simulink model "Twin_Builder"  (R2026a)
settings: Solver=VariableStepAuto  StopTime=simTime  FixedStep=Ts/60  RelTol=1e-2
values from neighbouring files (symbols this model uses):
  ac = log(9)/tr    [Run_Twin.m]
  as = 0.08 * ac    [Run_Twin.m]
  ath = 0.25 * as    [Run_Twin.m]
  B = 0.00001    (= 1e-05)    [Run_Twin.m]
  BEMFD_FEA_PerHz = InterpFEA_Data_ForSimulink(FEA_Data.BackEMFD_perHz, IS_FEA, IEA_FEA, IS_Interp, IEA_Interp)    [Run_Twin.m]
  BEMFQ_FEA_PerHz = InterpFEA_Data_ForSimulink(FEA_Data.BackEMFQ_perHz, IS_FEA, IEA_FEA, IS_Interp, IEA_Interp)    [Run_Twin.m]
  CondLoss_Inv = zeros([length(IS_Interp), size(FEA_Data.ConductionLoss, [2 3] ) ])    [Run_Twin.m]
  CopperLoss_FEA = InterpFEA_Data_ForSimulink(FEA_Data.CopperLosses, IS_FEA, IEA_FEA, IS_Interp, IEA_Interp)    [Run_Twin.m]
  DriveMethod = 1    [Run_Twin.m]
  EnvTorque_FW = interp1(Speed_full, Env_full, Speed_Vec, 'pchip', 'extrap')    [Run_Twin.m]
  f_sw = 10e3    (= 10000)    [Run_Twin.m]
  FEA_Data = LoadData.(FieldData{1})    [Run_Twin.m]
  FILTER_COEFF = 0.23    [Run_Twin.m]
  FluxD_FEA = InterpFEA_Data_ForSimulink(FEA_Data.FluxD, IS_FEA, IEA_FEA, IS_Interp, IEA_Interp)    [Run_Twin.m]
  FluxQ_FEA = InterpFEA_Data_ForSimulink(FEA_Data.FluxQ, IS_FEA, IEA_FEA, IS_Interp, IEA_Interp)    [Run_Twin.m]
  FrictLoss_FEA = squeeze( FEA_Data.FrictLosses(1,1,:) )    [Run_Twin.m]
  GateLoss_Inv = zeros([length(IS_Interp), size(FEA_Data.ConductionLoss, [2 3] ) ])    [Run_Twin.m]
  IDcore_FEA = InterpFEA_Data_ForSimulink(FEA_Data.IDc, IS_FEA, IEA_FEA, IS_Interp, IEA_Interp)    [Run_Twin.m]
  IEA_FEA = IEA_Interp    [Run_Twin.m]
  IQcore_FEA = InterpFEA_Data_ForSimulink(FEA_Data.IQc, IS_FEA, IEA_FEA, IS_Interp, IEA_Interp)    [Run_Twin.m]
  IronLoss_FEA = InterpFEA_Data_ForSimulink(FEA_Data.IronLosses,   IS_FEA, IEA_FEA, IS_Interp, IEA_Interp)    [Run_Twin.m]
  Is_Amp = 40    [Run_Twin.m]
  IS_FEA = IS_Interp    [Run_Twin.m]
  J = FEA_Data.Jinertia    [Run_Twin.m]
  J_Control = FEA_Data.Jinertia    [Run_Twin.m]
  LD_FEA = InterpFEA_Data_ForSimulink(FEA_Data.LD, IS_FEA, IEA_FEA, IS_Interp, IEA_Interp)    [Run_Twin.m]
  LD_Single = mean(LD_FEA, 'all')    [Run_Twin.m]
  LQ_FEA = InterpFEA_Data_ForSimulink(FEA_Data.LQ, IS_FEA, IEA_FEA, IS_Interp, IEA_Interp)    [Run_Twin.m]
  LQ_Single = mean(LQ_FEA, 'all')    [Run_Twin.m]
  MagnetLoss_FEA = InterpFEA_Data_ForSimulink(FEA_Data.MagnetLosses, IS_FEA, IEA_FEA, IS_Interp, IEA_Interp)    [Run_Twin.m]
  MaxSpeed = max(Speed_Vec)    [Run_Twin.m]
  MaxTe = max(Torque_FEA, [], 'all')    [Run_Twin.m]
  ModStrategy = 1    [Run_Twin.m]
  PMFlux_FEA = interp1(IS_FEA, squeeze( FEA_Data.FluxD(:,IEA_FEA == 90, :) ), IS_Interp, 'pchip' )    [Run_Twin.m]
  PMFlux_Single = mean( PMFlux_FEA, 'all' )    [Run_Twin.m]
  PMT_ID = round( F_ID(PMT_grid, Speed_grid), 2)    [Run_Twin.m]
  PMT_IQ = round( F_IQ(PMT_grid, Speed_grid), 2)    [Run_Twin.m]
  PMT_Vec = linspace(0,   100,   InterpSamples)    [Run_Twin.m]
  PolePair = FEA_Data.Poles / 2    [Run_Twin.m]
  PPR = 1024    [Run_Twin.m]
  ProxiLoss_FEA = InterpFEA_Data_ForSimulink(FEA_Data.ProxiLosses,  IS_FEA, IEA_FEA, IS_Interp, IEA_Interp)    [Run_Twin.m]
  Rcore_FEA = InterpFEA_Data_ForSimulink(FEA_Data.Rcore, IS_FEA, IEA_FEA, IS_Interp, IEA_Interp)    [Run_Twin.m]
  RDC = squeeze( Rseries_FEA(1,1,1) )    [Run_Twin.m]
  RefSpeed = [50, 400, 250, 500, 400]    [Run_Twin.m]
  RefTheta = [50, 0, 140, 300, -50]    [Run_Twin.m]
  Rseries_FEA = InterpFEA_Data_ForSimulink(FEA_Data.Rs,    IS_FEA, IEA_FEA, IS_Interp, IEA_Interp)    [Run_Twin.m]
  ShafthLoad = [10, 25, 3, 8, 10]    [Run_Twin.m]
  simTime = mechThetaTarget / wMechTarget    [Run_Twin.m]
  Speed_FEA = FEA_Data.Speed_vec    [Run_Twin.m]
  Speed_Vec = linspace(min(Speed_full), max(Speed_full), InterpSamples)    [Run_Twin.m]
  speedTarget = 200    [Run_Twin.m]
  SR_FEA = FEA_Data.SynchAngle    [Run_Twin.m]
  SwitchLoss_Inv = zeros([length(IS_Interp), size(FEA_Data.ConductionLoss, [2 3] ) ])    [Run_Twin.m]
  Tdt = 0.3 * 1e-6    (= 3e-07)    [Run_Twin.m]
  Throttle = 45    [Run_Twin.m]
  Times = [0, 0.2, 0.4, 0.6, 0.8] * simTime    [Run_Twin.m]
  Torque_FEA = InterpFEA_Data_ForSimulink(FEA_Data.TorqueFEA, IS_FEA, IEA_FEA, IS_Interp, IEA_Interp)    [Run_Twin.m]
  Ts = 1/f_sw    (= 0.0001)    [Run_Twin.m]
  Ts_Sp = 2 * Ts    (= 0.0002)    [Run_Twin.m]
  Vdc = 56    [Run_Twin.m]
  Vs_pu = 0.98    [Run_Twin.m]
  WindageLoss_FEA = squeeze( FEA_Data.WindLosses(1,1,:) )    [Run_Twin.m]
undefined symbols (not defined in the file or in its folder): DiscIntNeverNeededParam, feNom, mf, OverMod, PMT_Speed, SimData, Tables
libraries: simulink x14, ee_lib x11, simulink_extras x7, eeTransforms x6, fl_lib x6, eeGeneralControl x4, spsMeanLib x2, dspxfrm3 x1
(part 2 of 3)

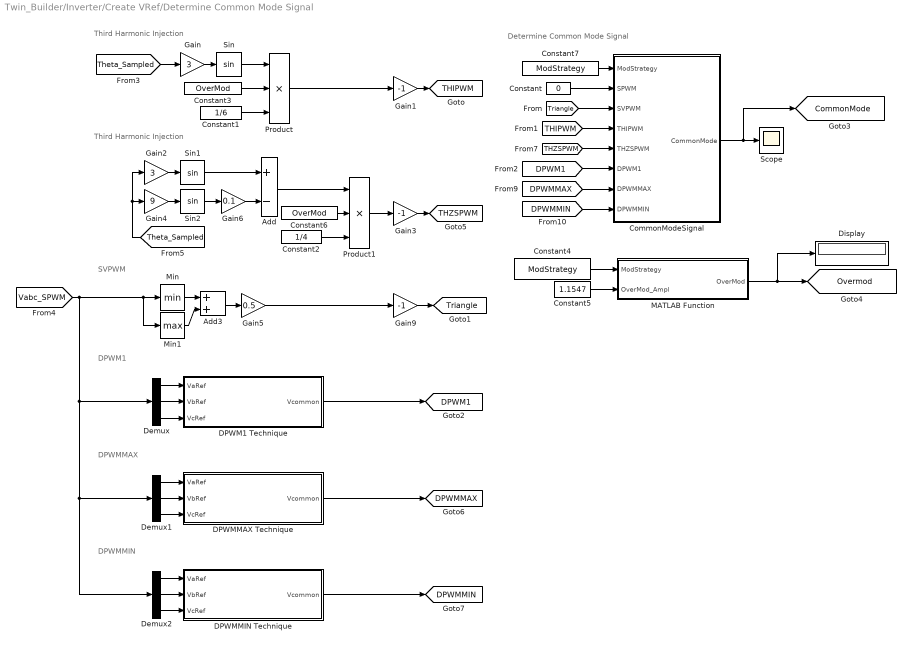
== system Twin_Builder/Inverter/Create VRef/Determine Common Mode Signal ==
  note: SVPWM
  note: Third Harmonic Injection
  note: Determine Common Mode Signal
  note: DPWM1
  note: Third Harmonic Injection
  note: DPWMMAX
  note: DPWMMIN
  Add : Sum  Inputs=+-
  Add3 : Sum
  CommonModeSignal : MATLAB Function  TreatAsAtomicUnit=on
  Constant : Constant  Value=0
  Constant1 : Constant  Value=1/6  SampleTime=0
  Constant2 : Constant  Value=1/4  SampleTime=0
  Constant3 : Constant  Value=OverMod  SampleTime=0
  Constant4 : Constant  Value=ModStrategy  SampleTime=0
  Constant5 : Constant  Value=1.1547  SampleTime=0
  Constant6 : Constant  Value=OverMod  SampleTime=0
  Constant7 : Constant  Value=ModStrategy  SampleTime=0
  DPWM1 Technique : MATLAB Function  TreatAsAtomicUnit=on
  DPWMMAX Technique : MATLAB Function  TreatAsAtomicUnit=on
  DPWMMIN Technique : MATLAB Function  TreatAsAtomicUnit=on
  Demux : Demux  Outputs=3
  Demux1 : Demux  Outputs=3
  Demux2 : Demux  Outputs=3
  Display : Display
  Gain : Gain  Gain=3
  Gain1 : Gain  Gain=-1
  Gain2 : Gain  Gain=3
  Gain3 : Gain  Gain=-1
  Gain4 : Gain  Gain=9
  Gain5 : Gain  Gain=0.5
  Gain6 : Gain  Gain=0.1
  Gain9 : Gain  Gain=-1
  MATLAB Function : MATLAB Function  TreatAsAtomicUnit=on
  Min : MinMax
  Min1 : MinMax  Function=max
  Product : Product  Inputs=3
  Product1 : Product  Inputs=3
  Scope : Scope
      settings: ActiveDisplayYMinimum=-0.35295  ActiveDisplayYMaximum=0.35321
  Sin : Trigonometry
  Sin1 : Trigonometry
  Sin2 : Trigonometry
  tag scope: CommonMode=global, DPWM1=global, DPWMMAX=global, DPWMMIN=global, Overmod=global, THIPWM=global, THZSPWM=global, Triangle=global
  wires:
  Constant/1 -> CommonModeSignal/2(SPWM)
  Min/1 -> Add3/1
  Gain9/1 -> [Triangle]
  Gain5/1 -> Gain9/1
  Add3/1 -> Gain5/1
  Min1/1 -> Add3/2
  Constant7/1 -> CommonModeSignal/1(ModStrategy)
  [Triangle] -> CommonModeSignal/3(SVPWM)
  [THIPWM] -> CommonModeSignal/4(THIPWM)
  DPWM1 Technique/1(Vcommon) -> [DPWM1]
  Demux/1 -> DPWM1 Technique/1(VaRef)
  Demux/2 -> DPWM1 Technique/2(VbRef)
  Demux/3 -> DPWM1 Technique/3(VcRef)
  CommonModeSignal/1(CommonMode) -> [CommonMode], Scope/1
  [Theta_Sampled] -> Gain/1
  Gain/1 -> Sin/1
  Sin/1 -> Product/1
  Constant3/1 -> Product/2
  Constant1/1 -> Product/3
  Product/1 -> Gain1/1
  Constant4/1 -> MATLAB Function/1(ModStrategy)
  Constant5/1 -> MATLAB Function/2(OverMod_Ampl)
  MATLAB Function/1(OverMod) -> Display/1, [Overmod]
  Gain1/1 -> [THIPWM]
  Gain2/1 -> Sin1/1
  [Theta_Sampled] -> Gain2/1, Gain4/1
  Constant6/1 -> Product1/2
  Gain4/1 -> Sin2/1
  Product1/1 -> Gain3/1
  Gain3/1 -> [THZSPWM]
  Sin2/1 -> Gain6/1
  Sin1/1 -> Add/1
  Gain6/1 -> Add/2
  Add/1 -> Product1/1
  [DPWM1] -> CommonModeSignal/6(DPWM1)
  [THZSPWM] -> CommonModeSignal/5(THZSPWM)
  Constant2/1 -> Product1/3
  DPWMMAX Technique/1(Vcommon) -> [DPWMMAX]
  Demux1/1 -> DPWMMAX Technique/1(VaRef)
  Demux1/2 -> DPWMMAX Technique/2(VbRef)
  Demux1/3 -> DPWMMAX Technique/3(VcRef)
  [DPWMMAX] -> CommonModeSignal/7(DPWMMAX)
  [DPWMMIN] -> CommonModeSignal/8(DPWMMIN)
  Demux2/1 -> DPWMMIN Technique/1(VaRef)
  Demux2/3 -> DPWMMIN Technique/3(VcRef)
  Demux2/2 -> DPWMMIN Technique/2(VbRef)
  DPWMMIN Technique/1(Vcommon) -> [DPWMMIN]
  [Vabc_SPWM] -> Demux/1, Demux1/1, Demux2/1, Min1/1, Min/1

== system Twin_Builder/Inverter/Create VRef/Finalize References ==
  note: Wrap References to [0,1] and saturate them
  Vabc_Ref : Inport
  Add : Sum
  Constant1 : Constant  Value=0  SampleTime=0
  Constant2 : Constant  Value=0.5  SampleTime=0
  Constant3 : Constant  SampleTime=0
  Demux : Demux  Outputs=3
  Divide1 : Product  Inputs=*/
  Gain3 : Gain  Gain=0.5
  Max : MinMax  Function=max  Inputs=4
  Max1 : MinMax  Function=max  Inputs=2
  Vabc_Ref_Final : Outport
  wires:
  Constant2/1 -> Add/2
  Gain3/1 -> Add/1
  Vabc_Ref/1 -> Gain3/1
  Demux/3 -> Max/3
  Constant3/1 -> Max/4
  Demux/1 -> Max/1
  Demux/2 -> Max/2
  Max/1 -> Divide1/2
  Add/1 -> Divide1/1, Demux/1
  Divide1/1 -> Max1/1
  Max1/1 -> Vabc_Ref_Final/1
  Constant1/1 -> Max1/2

== system Twin_Builder/PMSM /LUTS/QEP  ==
  theta : Inport
  Abs1 : Abs  SaturateOnIntegerOverflow=off
  Constant1 : Constant  Value=PolePair
  Constant3 : Constant  Value=Ts_Sp
  Constant5 : Constant  Value=PolePair
  Constant6 : Constant  Value=FILTER_COEFF
  Constant8 : Constant  Value=PPR
  Divide2 : Product  Inputs=*/
  Product : Product
  "Quantize Electrical Theta " : MATLAB Function  TreatAsAtomicUnit=on
  Sample θ : MATLAB Function  TreatAsAtomicUnit=on
  Scope : Scope
      settings: ActiveDisplayYMinimum=-0.78520641579896233  ActiveDisplayYMaximum=7.0668577421906633
  Terminator1 : Terminator
  Terminator2 : Terminator
  omega2rpm2 : Gain  Gain=60/(2*pi)
  theta_sampled : Outport
  Omegae : Outport  Port=2
  Speed : Outport  Port=3
  wires:
  omega2rpm2/1 -> Abs1/1
  Constant6/1 -> Sample θ/3(FILTER_COEFF)
  Abs1/1 -> Speed/1
  Sample θ/2(delta_theta) -> Terminator2/1
  Constant3/1 -> Sample θ/2(Ts)
  Constant1/1 -> Divide2/2
  Sample θ/1(omega) -> Divide2/1
  Divide2/1 -> Product/2, omega2rpm2/1
  Constant8/1 -> "Quantize Electrical Theta "/2(PPR)
  theta/1 -> "Quantize Electrical Theta "/1(theta_w)
  "Quantize Electrical Theta "/2(Count) -> Terminator1/1
  "Quantize Electrical Theta "/1(Theta_mcu) -> Scope/1, theta_sampled/1, Sample θ/1(theta)
  Constant5/1 -> Product/1
  Product/1 -> Omegae/1

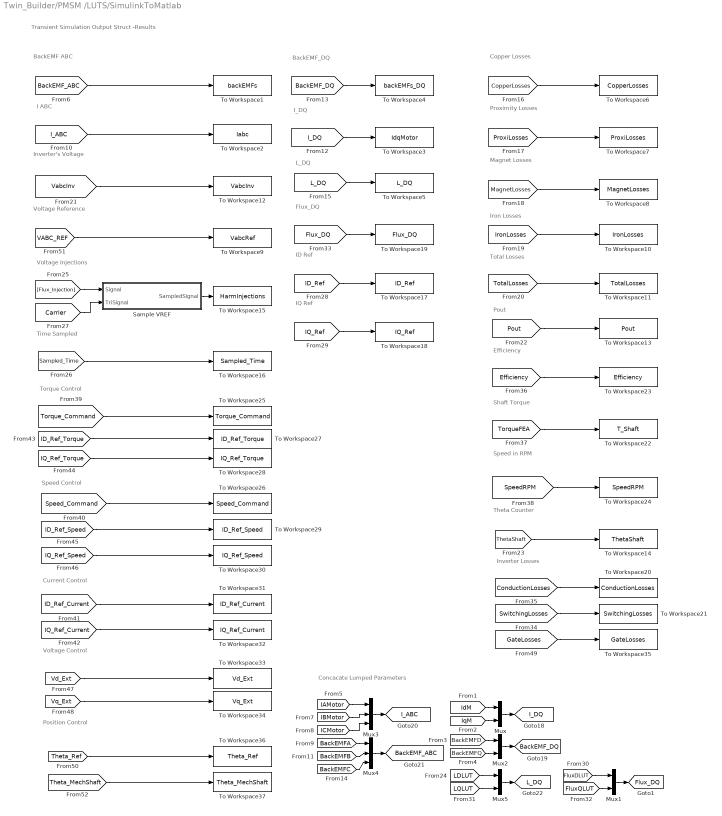
== system Twin_Builder/PMSM /LUTS/SimulinkToMatlab ==
  note: Voltage Reference
  note: Transient Simulation Output Struct -Results
  note: BackEMF ABC
  note: I_DQ
  note: BackEMF_DQ
  note: L_DQ
  note: Copper Losses
  note: Proximity Losses
  note: Magnet Losses
  note: Iron Losses
  note: Total Losses
  note: Inverter's Voltage
  note: Pout
  note: Theta Counter
  note: Voltage Injections
  note: Time Sampled
  note: ID Ref
  note: IQ Ref
  note: Efficiency
  note: Concacate Lumped Parameters
  note: I ABC
  note: Flux_DQ
  note: Inverter Losses
  note: Shaft Torque
  note: Speed in RPM
  note: Torque Control
  note: Speed Control
  note: Current Control
  note: Voltage Control
  note: Position Control
  Mux{,1..2,5} (4 alike) : Mux  Inputs=2
  Mux3 : Mux  Inputs=3
  Mux4 : Mux  Inputs=3
  Sample VREF : MATLAB Function  TreatAsAtomicUnit=on
  To Workspace1 : ToWorkspace  VariableName=backEMFs  SampleTime=-1
  To Workspace10 : ToWorkspace  VariableName=IronLosses  SampleTime=-1
  To Workspace11 : ToWorkspace  VariableName=TotalLosses  SampleTime=-1
  To Workspace12 : ToWorkspace  VariableName=VabcInv  SampleTime=-1
  To Workspace13 : ToWorkspace  VariableName=Pout  SampleTime=-1
  To Workspace14 : ToWorkspace  VariableName=ThetaShaft  SampleTime=-1
  To Workspace15 : ToWorkspace  VariableName=HarmInjections  SampleTime=-1
  To Workspace16 : ToWorkspace  VariableName=Sampled_Time  SampleTime=-1
  To Workspace17 : ToWorkspace  VariableName=ID_Ref  SampleTime=-1
  To Workspace18 : ToWorkspace  VariableName=IQ_Ref  SampleTime=-1
  To Workspace19 : ToWorkspace  VariableName=Flux_DQ  SampleTime=-1
  To Workspace2 : ToWorkspace  VariableName=Iabc  SampleTime=-1
  To Workspace20 : ToWorkspace  VariableName=ConductionLosses  SampleTime=-1
  To Workspace21 : ToWorkspace  VariableName=SwitchingLosses  SampleTime=-1
  To Workspace22 : ToWorkspace  VariableName=T_Shaft  SampleTime=-1
  To Workspace23 : ToWorkspace  VariableName=Efficiency  SampleTime=-1
  To Workspace24 : ToWorkspace  VariableName=SpeedRPM  SampleTime=-1
  To Workspace25 : ToWorkspace  VariableName=Torque_Command  SampleTime=-1
  To Workspace26 : ToWorkspace  VariableName=Speed_Command  SampleTime=-1
  To Workspace27 : ToWorkspace  VariableName=ID_Ref_Torque  SampleTime=-1
  To Workspace28 : ToWorkspace  VariableName=IQ_Ref_Torque  SampleTime=-1
  To Workspace29 : ToWorkspace  VariableName=ID_Ref_Speed  SampleTime=-1
  To Workspace3 : ToWorkspace  VariableName=IdqMotor  SampleTime=-1
  To Workspace30 : ToWorkspace  VariableName=IQ_Ref_Speed  SampleTime=-1
  To Workspace31 : ToWorkspace  VariableName=ID_Ref_Current  SampleTime=-1
  To Workspace32 : ToWorkspace  VariableName=IQ_Ref_Current  SampleTime=-1
  To Workspace33 : ToWorkspace  VariableName=Vd_Ext  SampleTime=-1
  To Workspace34 : ToWorkspace  VariableName=Vq_Ext  SampleTime=-1
  To Workspace35 : ToWorkspace  VariableName=GateLosses  SampleTime=-1
  To Workspace36 : ToWorkspace  VariableName=Theta_Ref  SampleTime=-1
  To Workspace37 : ToWorkspace  VariableName=Theta_MechShaft  SampleTime=-1
  To Workspace4 : ToWorkspace  VariableName=backEMFs_DQ  SampleTime=-1
  To Workspace5 : ToWorkspace  VariableName=L_DQ  SampleTime=-1
  To Workspace6 : ToWorkspace  VariableName=CopperLosses  SampleTime=-1
  To Workspace7 : ToWorkspace  VariableName=ProxiLosses  SampleTime=-1
  To Workspace8 : ToWorkspace  VariableName=MagnetLosses  SampleTime=-1
  To Workspace9 : ToWorkspace  VariableName=VabcRef  SampleTime=-1
  tag scope: BackEMF_ABC=global, BackEMF_DQ=global, Flux_DQ=global, I_ABC=global, I_DQ=global, L_DQ=global
  wires:
  [ThetaShaft] -> To Workspace14/1
  [BackEMF_DQ] -> To Workspace4/1
  [VabcInv] -> To Workspace12/1
  [I_DQ] -> To Workspace3/1
  [Efficiency] -> To Workspace23/1
  [CopperLosses] -> To Workspace6/1
  [BackEMF_ABC] -> To Workspace1/1
  [VABC_REF] -> To Workspace9/1
  [MagnetLosses] -> To Workspace8/1
  [ProxiLosses] -> To Workspace7/1
  [Flux_Injection] -> Sample VREF/1(Signal)
  Sample VREF/1(SampledSignal) -> To Workspace15/1
  [Pout] -> To Workspace13/1
  [TotalLosses] -> To Workspace11/1
  [IQ_Ref] -> To Workspace18/1
  [Carrier] -> Sample VREF/2(TriSignal)
  [IronLosses] -> To Workspace10/1
  [ID_Ref] -> To Workspace17/1
  [L_DQ] -> To Workspace5/1
  [Sampled_Time] -> To Workspace16/1
  [BackEMFC] -> Mux4/3
  [BackEMFA] -> Mux4/1
  Mux4/1 -> [BackEMF_ABC]
  [BackEMFB] -> Mux4/2
  [LQLUT] -> Mux5/2
  Mux3/1 -> [I_ABC]
  Mux/1 -> [I_DQ]
  [LDLUT] -> Mux5/1
  [IdM] -> Mux/1
  [IBMotor] -> Mux3/2
  [IAMotor] -> Mux3/1
  [ICMotor] -> Mux3/3
  Mux5/1 -> [L_DQ]
  [IqM] -> Mux/2
  Mux2/1 -> [BackEMF_DQ]
  [BackEMFQ] -> Mux2/2
  [BackEMFD] -> Mux2/1
  [I_ABC] -> To Workspace2/1
  [FluxDLUT] -> Mux1/1
  Mux1/1 -> [Flux_DQ]
  [FluxQLUT] -> Mux1/2
  [Flux_DQ] -> To Workspace19/1
  [ConductionLosses] -> To Workspace20/1
  [SwitchingLosses] -> To Workspace21/1
  [TorqueFEA] -> To Workspace22/1
  [SpeedRPM] -> To Workspace24/1
  [Torque_Command] -> To Workspace25/1
  [Speed_Command] -> To Workspace26/1
  [ID_Ref_Torque] -> To Workspace27/1
  [IQ_Ref_Torque] -> To Workspace28/1
  [ID_Ref_Speed] -> To Workspace29/1
  [IQ_Ref_Speed] -> To Workspace30/1
  [ID_Ref_Current] -> To Workspace31/1
  [IQ_Ref_Current] -> To Workspace32/1
  [Vd_Ext] -> To Workspace33/1
  [Vq_Ext] -> To Workspace34/1
  [GateLosses] -> To Workspace35/1
  [Theta_Ref] -> To Workspace36/1
  [Theta_MechShaft] -> To Workspace37/1

== system Twin_Builder/PMSM /LUTS/TorqueInduced from Fluxes ==
  note: Torque with Fluxes
  Gain1 : Gain  Gain=3*PolePair/2
  Product3 : Product
  Product4 : Product
  Sum2 : Sum  Inputs=|+-
  tag scope: Te=global
  wires:
  [FluxDLUT] -> Product3/1
  [IqM] -> Product3/2
  [FluxQLUT] -> Product4/1
  [IdM] -> Product4/2
  Product3/1 -> Sum2/1
  Product4/1 -> Sum2/2
  Sum2/1 -> Gain1/1
  Gain1/1 -> [Te]

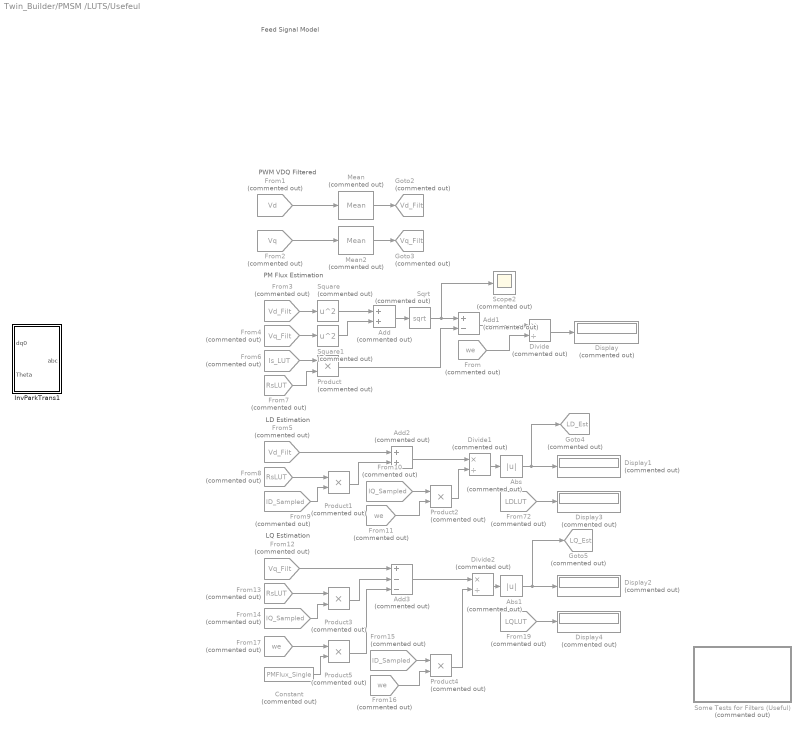
== system Twin_Builder/PMSM /LUTS/Usefeul ==
  note: PM Flux Estimation
  note: PWM VDQ Filtered
  note: LD Estimation
  note: LQ Estimation
  note: Feed Signal Model
  Abs : Abs  Commented=on  SaturateOnIntegerOverflow=off
  Abs1 : Abs  Commented=on  SaturateOnIntegerOverflow=off
  Add : Sum  Commented=on
  Add1 : Sum  Commented=on  Inputs=+-
  Add2 : Sum  Commented=on
  Add3 : Sum  Commented=on  Inputs=+--
  Constant : Constant  Commented=on  Value=PMFlux_Single  SampleTime=0
  Display{,1..4} (5 alike) : Display  Commented=on
  Divide : Product  Commented=on  Inputs=*/
  Divide1 : Product  Commented=on  Inputs=*/
  Divide2 : Product  Commented=on  Inputs=*/
  From{,11,16..17} (4 alike) : From  Commented=on  GotoTag=we  TagVisibility=global
  From1 : From  Commented=on  GotoTag=Vd  TagVisibility=global
  From10 : From  Commented=on  GotoTag=IQ_Sampled  TagVisibility=global
  From12 : From  Commented=on  GotoTag=Vq_Filt  TagVisibility=global
  From13 : From  Commented=on  GotoTag=RsLUT  TagVisibility=global
  From14 : From  Commented=on  GotoTag=IQ_Sampled  TagVisibility=global
  From15 : From  Commented=on  GotoTag=ID_Sampled  TagVisibility=global
  From19 : From  Commented=on  GotoTag=LQLUT  TagVisibility=global
  From2 : From  Commented=on  GotoTag=Vq  TagVisibility=global
  From3 : From  Commented=on  GotoTag=Vd_Filt  TagVisibility=global
  From4 : From  Commented=on  GotoTag=Vq_Filt  TagVisibility=global
  From5 : From  Commented=on  GotoTag=Vd_Filt  TagVisibility=global
  From6 : From  Commented=on  GotoTag=Is_LUT  TagVisibility=global
  From7 : From  Commented=on  GotoTag=RsLUT  TagVisibility=global
  From72 : From  Commented=on  GotoTag=LDLUT  TagVisibility=global
  From8 : From  Commented=on  GotoTag=RsLUT  TagVisibility=global
  From9 : From  Commented=on  GotoTag=ID_Sampled  TagVisibility=global
  Goto2 : Goto  Commented=on  GotoTag=Vd_Filt  TagVisibility=global
  Goto3 : Goto  Commented=on  GotoTag=Vq_Filt  TagVisibility=global
  Goto4 : Goto  Commented=on  GotoTag=LD_Est  TagVisibility=global
  Goto5 : Goto  Commented=on  GotoTag=LQ_Est  TagVisibility=global
  InvParkTrans1 : Subsystem
  Mean : spsMeanLib/Mean  Commented=on  Freq=60  Vinit=0  Ts=0
  Mean2 : spsMeanLib/Mean  Commented=on  Freq=60  Vinit=0  Ts=0
  Product{,1..5} (6 alike) : Product  Commented=on
  Scope2 : Scope  Commented=on
      settings: ActiveDisplayYMinimum=-0.82581  ActiveDisplayYMaximum=7.43229
  Some Tests for Filters (Useful) : Subsystem  Commented=on
  Sqrt : Sqrt  Commented=on
  Square : Math  Commented=on  Operator=square
  Square1 : Math  Commented=on  Operator=square
  wires:
  Add/1 -> Sqrt/1
  Square1/1 -> Add/2
  Square/1 -> Add/1
  From6/1 -> Product/1
  From7/1 -> Product/2
  Product/1 -> Add1/2
  Add1/1 -> Divide/1
  From/1 -> Divide/2
  Divide/1 -> Display/1
  Sqrt/1 -> Scope2/1, Add1/1
  From3/1 -> Square/1
  From4/1 -> Square1/1
  From2/1 -> Mean2/1
  From1/1 -> Mean/1
  Mean/1 -> Goto2/1
  Mean2/1 -> Goto3/1
  From5/1 -> Add2/1
  From9/1 -> Product1/2
  From8/1 -> Product1/1
  Product1/1 -> Add2/2
  From10/1 -> Product2/1
  From11/1 -> Product2/2
  Add2/1 -> Divide1/1
  Product2/1 -> Divide1/2
  Divide1/1 -> Abs/1
  From14/1 -> Product3/2
  From13/1 -> Product3/1
  From12/1 -> Add3/1
  Product3/1 -> Add3/2
  From16/1 -> Product4/2
  From15/1 -> Product4/1
  From17/1 -> Product5/1
  Constant/1 -> Product5/2
  Product5/1 -> Add3/3
  Add3/1 -> Divide2/1
  Product4/1 -> Divide2/2
  Divide2/1 -> Abs1/1
  From72/1 -> Display3/1
  From19/1 -> Display4/1
  Abs/1 -> Display1/1, Goto4/1
  Abs1/1 -> Display2/1, Goto5/1

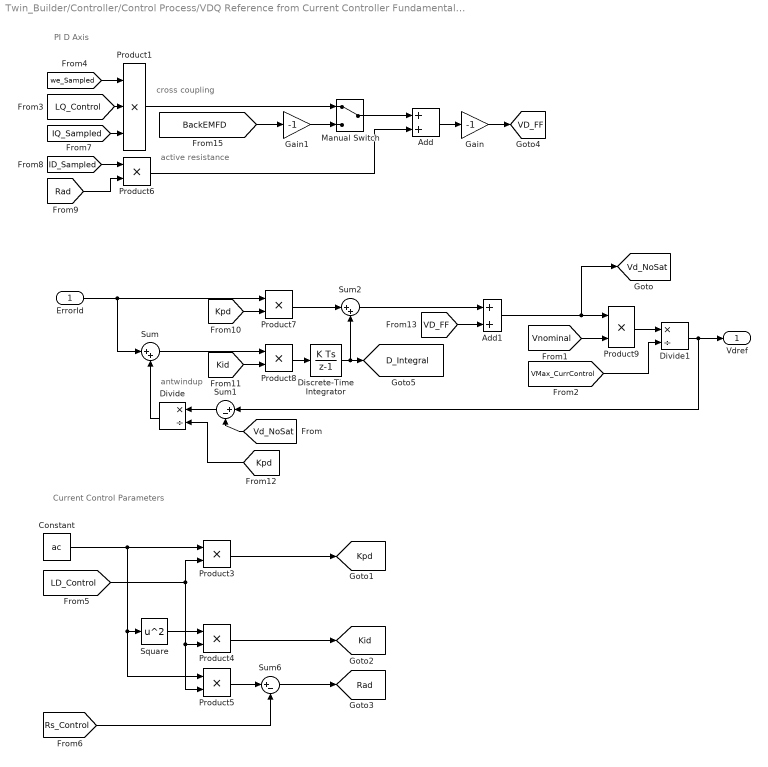
== system Twin_Builder/Controller/Control Process/VDQ Reference from Current Controller Fundamental/CurrentControlD ==
  note: active resistance
  note: cross coupling
  note: Current Control Parameters
  note: PI D Axis
  note: antwindup
  ErrorId : Inport
  Add : Sum
  Add1 : Sum
  Constant : Constant  Value=ac  SampleTime=0
  Discrete-Time Integrator : DiscreteIntegrator  SampleTime=Ts  ICPrevOutput=DiscIntNeverNeededParam  ICPrevScaledInput=DiscIntNeverNeededParam
  Divide : Product  Inputs=*/
  Divide1 : Product  Inputs=*/
  Gain : Gain  Gain=-1
  Gain1 : Gain  Gain=-1
  Manual Switch : ManualSwitch
  Product1 : Product  Inputs=3
  Product{3..9} (7 alike) : Product
  Square : Math  Operator=square
  Sum : Sum  Inputs=|++
  Sum1 : Sum  Inputs=|+-
  Sum2 : Sum  Inputs=|++
  Sum6 : Sum  Inputs=|+-
  Vdref : Outport
  tag scope: D_Integral=global, Kid=global, Kpd=global, Rad=global, VD_FF=global, Vd_NoSat=global
  wires:
  Sum/1 -> Product8/1
  Product7/1 -> Sum2/1
  ErrorId/1 -> Sum/1, Product7/1
  Product8/1 -> Discrete-Time Integrator/1
  Product6/1 -> Add/2
  Sum2/1 -> Add1/1
  Discrete-Time Integrator/1 -> [D_Integral], Sum2/2
  Product3/1 -> [Kpd]
  Square/1 -> Product4/1
  Constant/1 -> Product3/1, Product5/1, Square/1
  Product5/1 -> Sum6/1
  Sum6/1 -> [Rad]
  [Rad] -> Product6/2
  [Kpd] -> Product7/2
  [Kid] -> Product8/2
  Sum1/1 -> Divide/1
  Divide/1 -> Sum/2
  [Kpd] -> Divide/2
  Product4/1 -> [Kid]
  [Rs_Control] -> Sum6/2
  [LD_Control] -> Product3/2, Product5/2, Product4/2
  [Vnominal] -> Product9/2
  Product9/1 -> Divide1/1
  [VMax_CurrControl] -> Divide1/2
  Divide1/1 -> Vdref/1, Sum1/1
  [ID_Sampled] -> Product6/1
  [we_Sampled] -> Product1/1
  [LQ_Control] -> Product1/2
  [IQ_Sampled] -> Product1/3
  [Vd_NoSat] -> Sum1/2
  Add/1 -> Gain/1
  Gain/1 -> [VD_FF]
  Add1/1 -> [Vd_NoSat], Product9/1
  [VD_FF] -> Add1/2
  Manual Switch/1 -> Add/1
  Product1/1 -> Manual Switch/1
  [BackEMFD] -> Gain1/1
  Gain1/1 -> Manual Switch/2

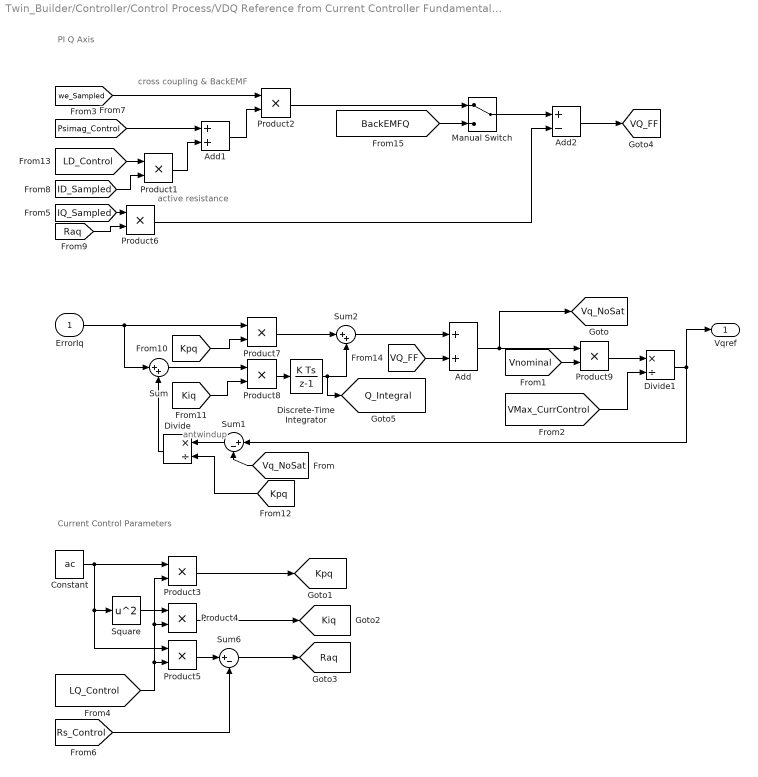
== system Twin_Builder/Controller/Control Process/VDQ Reference from Current Controller Fundamental/CurrentControlQ ==
  note: active resistance
  note: cross coupling & BackEMF
  note: Current Control Parameters
  note: PI Q Axis
  note: antwindup
  ErrorIq : Inport
  Add : Sum
  Add1 : Sum
  Add2 : Sum  Inputs=+-
  Constant : Constant  Value=ac
  Discrete-Time Integrator : DiscreteIntegrator  SampleTime=Ts  ICPrevOutput=DiscIntNeverNeededParam  ICPrevScaledInput=DiscIntNeverNeededParam
  Divide : Product  Inputs=*/
  Divide1 : Product  Inputs=*/
  Manual Switch : ManualSwitch
  Product{1..9} (9 alike) : Product
  Square : Math  Operator=square
  Sum : Sum  Inputs=|++
  Sum1 : Sum  Inputs=|+-
  Sum2 : Sum  Inputs=|++
  Sum6 : Sum  Inputs=|+-
  Vqref : Outport
  tag scope: Kiq=global, Kpq=global, Q_Integral=global, Raq=global, VQ_FF=global, Vq_NoSat=global
  wires:
  Sum/1 -> Product8/1
  Product7/1 -> Sum2/1
  ErrorIq/1 -> Product7/1, Sum/1
  Product8/1 -> Discrete-Time Integrator/1
  Discrete-Time Integrator/1 -> Sum2/2, [Q_Integral]
  Product3/1 -> [Kpq]
  Square/1 -> Product4/1
  Constant/1 -> Product5/1, Square/1, Product3/1
  Product5/1 -> Sum6/1
  Sum6/1 -> [Raq]
  [Raq] -> Product6/2
  [Kpq] -> Product7/2
  [Kiq] -> Product8/2
  Sum1/1 -> Divide/1
  Divide/1 -> Sum/2
  [Kpq] -> Divide/2
  Product4/1 -> [Kiq]
  [Rs_Control] -> Sum6/2
  [LQ_Control] -> Product3/2, Product4/2, Product5/2
  [Vnominal] -> Product9/2
  [VMax_CurrControl] -> Divide1/2
  Add/1 -> [Vq_NoSat], Product9/1
  Product9/1 -> Divide1/1
  Divide1/1 -> Vqref/1, Sum1/1
  [ID_Sampled] -> Product1/2
  [IQ_Sampled] -> Product6/1
  [LD_Control] -> Product1/1
  Product1/1 -> Add1/2
  [Psimag_Control] -> Add1/1
  [we_Sampled] -> Product2/1
  Add1/1 -> Product2/2
  Product6/1 -> Add2/2
  Add2/1 -> [VQ_FF]
  [Vq_NoSat] -> Sum1/2
  Sum2/1 -> Add/1
  [VQ_FF] -> Add/2
  Product2/1 -> Manual Switch/1
  Manual Switch/1 -> Add2/1
  [BackEMFQ] -> Manual Switch/2

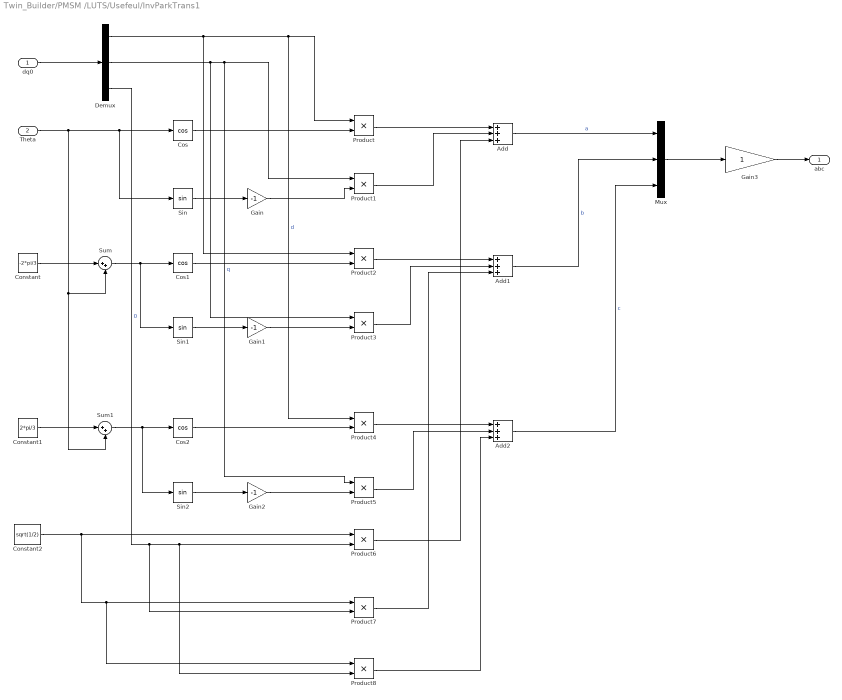
== system Twin_Builder/PMSM /LUTS/Usefeul/InvParkTrans1 ==
  dq0 : Inport
  Theta : Inport  Port=2
  Add : Sum  Inputs=+++
  Add1 : Sum  Inputs=+++
  Add2 : Sum  Inputs=+++
  Constant : Constant  Value=-2*pi/3  SampleTime=0
  Constant1 : Constant  Value=2*pi/3  SampleTime=0
  Constant2 : Constant  Value=sqrt(1/2)  SampleTime=0
  Cos : Trigonometry  Operator=cos
  Cos1 : Trigonometry  Operator=cos
  Cos2 : Trigonometry  Operator=cos
  Demux : Demux  Outputs=3
  Gain : Gain  Gain=-1
  Gain1 : Gain  Gain=-1
  Gain2 : Gain  Gain=-1
  Gain3 : Gain
  Mux : Mux  Inputs=3
  Product{,1..8} (9 alike) : Product
  Sin : Trigonometry
  Sin1 : Trigonometry
  Sin2 : Trigonometry
  Sum : Sum  Inputs=|++
  Sum1 : Sum  Inputs=|++
  abc : Outport
  wires:
  Gain3/1 -> abc/1
  Mux/1 -> Gain3/1
  Add2/1 -> Mux/3  "c"
  Add1/1 -> Mux/2  "b"
  Add/1 -> Mux/1  "a"
  Product8/1 -> Add2/3
  Product5/1 -> Add2/2
  Gain2/1 -> Product5/2
  Sin2/1 -> Gain2/1
  Product4/1 -> Add2/1
  Product7/1 -> Add1/3
  Product3/1 -> Add1/2
  Gain1/1 -> Product3/2
  Sin1/1 -> Gain1/1
  Product2/1 -> Add1/1
  Product6/1 -> Add/3
  Demux/3 -> Product6/2, Product8/2, Product7/2  "0"
  Product1/1 -> Add/2
  Product/1 -> Add/1
  Constant2/1 -> Product6/1, Product7/1, Product8/1
  Demux/2 -> Product3/1, Product5/1, Product1/1  "q"
  Gain/1 -> Product1/2
  Sin/1 -> Gain/1
  Demux/1 -> Product2/1, Product/1, Product4/1  "d"
  Cos2/1 -> Product4/2
  Cos1/1 -> Product2/2
  Cos/1 -> Product/2
  dq0/1 -> Demux/1
  Sum/1 -> Cos1/1, Sin1/1
  Sum1/1 -> Cos2/1, Sin2/1
  Constant1/1 -> Sum1/1
  Constant/1 -> Sum/1
  Theta/1 -> Cos/1, Sin/1, Sum/2, Sum1/2

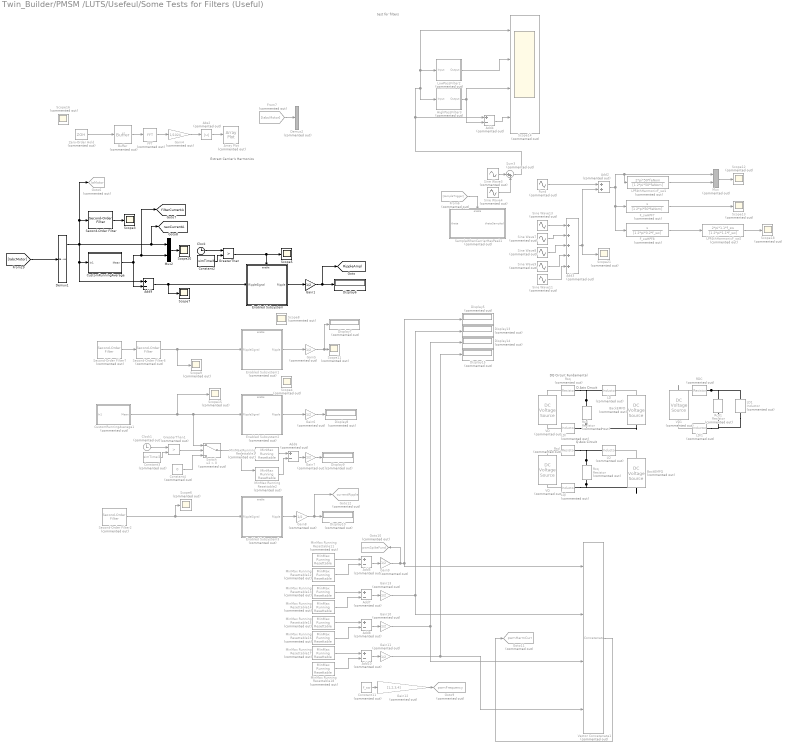
== system Twin_Builder/PMSM /LUTS/Usefeul/Some Tests for Filters (Useful) ==
  note: Extract Carrier's Harmonics
  note: test for filters
  note: D Axis Circuit
  note: DQ Circuit Fundamental
  note: Q Axis Circuit
  Abs2 : Abs  Commented=on  SaturateOnIntegerOverflow=off
  Add{4..8,10} (6 alike) : Sum  Commented=on  Inputs=+-
  Add2 : Sum  Commented=on
  Add3 : Sum  Commented=on  Inputs=+++++
  Add9 : Sum  Inputs=+-
  Array Plot : ArrayPlot  Commented=on  WindowPosition=[368.000000,182.000000,800.000000,500.000000,]  ScopeFrameLocation=window  PlotType=Stairs  PlotAsMagnitudePhase=on
  BackEMFD : ee_lib/Additional Components/SPICE Sources/DC Voltage Source  Commented=on  DC=0 V
  BackEMFQ : ee_lib/Additional Components/SPICE Sources/DC Voltage Source  Commented=on  DC=0 V
  Buffer : Buffer  Commented=on  N=1024  OutputFrames=off
  Clock : Clock
  Clock1 : Clock  Commented=on
  Constant11 : Constant  Commented=on  Value=f_sw  SampleTime=Ts
  Constant2 : Constant  Value=simTime/6  VectorParams1D=off
  Constant3 : Constant  Commented=on  Value=simTime/2  VectorParams1D=off
  Constant4 : Constant  Commented=on  Value=0  SampleTime=0
  CustomRunningAverage : Subsystem
  CustomRunningAverage1 : Subsystem  Commented=on
  Demux1 : Demux  Outputs=3
  Demux2 : Demux  Commented=on  Outputs=3
  Display{5,7..10,13..15} (8 alike) : Display  Commented=on
  Display6 : Display
  Enabled Subsystem : Subsystem  TreatAsAtomicUnit=on
  Enabled Subsystem1 : Subsystem  Commented=on  TreatAsAtomicUnit=on
  Enabled Subsystem2 : Subsystem  Commented=on  TreatAsAtomicUnit=on
  Enabled Subsystem3 : Subsystem  Commented=on  TreatAsAtomicUnit=on
  FFT : dspxfrm3/FFT  Commented=on  FFTImplementation=Auto  CompMethod=Table lookup  TableOpt=NEW  TableOptActive=Speed  BitRevOrder=off  Normalize=off  InheritFFTLength=on  FFTLength=64  WrapInput=on  roundingMode=Floor  overflowMode=off  firstCoeffDataTypeStr=Inherit: Same word length as input  firstCoeffLastDataTypeStr=Inherit: Same word length as input  outputMin=[]  outputMax=[]
  F_swHPF7 : TransferFcn  Commented=on  Numerator=[1 0]  Denominator=[1 2*pi*50*feNom]
  F_swHPF8 : TransferFcn  Commented=on  Numerator=[1 0]  Denominator=[1 2*pi*0.2*f_sw]
  From6 : From  Commented=on  GotoTag=sampleTrigger  TagVisibility=global
  From7 : From  Commented=on  GotoTag=IabcMotor  TagVisibility=global
  Fund : Sin  Commented=on  Amplitude=10  Frequency=feNom*2*pi  SampleTime=0
  Gain1 : Gain  Gain=1/2
  Gain{5..11,13} (8 alike) : Gain  Commented=on  Gain=1/2
  Gain12 : Gain  Commented=on  Gain=[1,2,3,4]
  Gain4 : Gain  Commented=on  Gain=1/1024
  Goto10 : Goto  Commented=on  GotoTag=pwmSpikeFund  TagVisibility=global
  Goto11 : Goto  Commented=on  GotoTag=pwmHarmCurr  TagVisibility=global
  Goto12 : Goto  Commented=on  GotoTag=currentRipple  TagVisibility=global
  Goto6 : Goto  Commented=on  GotoTag=IaMotor  TagVisibility=global
  Goto9 : Goto  Commented=on  GotoTag=pwmFrequency  TagVisibility=global
  GreaterThan : RelationalOperator  Operator=>  OutDataTypeStr=boolean  RndMeth=Simplest  InputSameDT=off
  GreaterThan1 : RelationalOperator  Commented=on  Operator=>  OutDataTypeStr=boolean  RndMeth=Simplest  InputSameDT=off
  HighPassFilter3 : Subsystem  Commented=on
  LD : ee_lib/Passive/Inductor  Commented=on  l=1e-6 H  enable_L_tol=ee.enum.toleranceApplication.none  L_tol=20  tol_distribution=ee.enum.toleranceDistribution.uniform  nSigma=4  r=0 Ohm  g=1e-9 1/Ohm  enable_operating_limits=ee.enum.enable.no  operating_limit_action=ee.enum.passive.reportOpLim.warn  max_working_current=1 A  power_rating=1 W  enable_faults=ee.enum.enable.no  fault_action=simscape.enum.assert.action.none  lambdaPercent=50  k_faulted=0.9999  turnsShort=ee.enum.passive.inductor.turnsShortOption.no  openCct=ee.enum.enable.no  groundShort=ee.enum.passive.inductor.groundShortOption.no  groundShortG=0 1/Ohm  tau_fault=1e-3 s  fault_trigger=ee.enum.faults.faultTrigger.temporal  t_fault=1 s  max_permissible_voltage=100 V  n_fail_on_voltage=1  max_permissible_current=1 A  t_fail_on_current=1 s  i_L_specify=off  i_L_priority=High  i_L=0 A  i_L_nominal_specify=off  i_L_nominal_value=1  i_L_nominal_unit=A  faulted_specify=off  faulted_priority=None  faulted=0
  LD1 : ee_lib/Passive/Inductor  Commented=on  l=1e-6 H  enable_L_tol=ee.enum.toleranceApplication.none  L_tol=20  tol_distribution=ee.enum.toleranceDistribution.uniform  nSigma=4  r=0 Ohm  g=1e-9 1/Ohm  enable_operating_limits=ee.enum.enable.no  operating_limit_action=ee.enum.passive.reportOpLim.warn  max_working_current=1 A  power_rating=1 W  enable_faults=ee.enum.enable.no  fault_action=simscape.enum.assert.action.none  lambdaPercent=50  k_faulted=0.9999  turnsShort=ee.enum.passive.inductor.turnsShortOption.no  openCct=ee.enum.enable.no  groundShort=ee.enum.passive.inductor.groundShortOption.no  groundShortG=0 1/Ohm  tau_fault=1e-3 s  fault_trigger=ee.enum.faults.faultTrigger.temporal  t_fault=1 s  max_permissible_voltage=100 V  n_fail_on_voltage=1  max_permissible_current=1 A  t_fail_on_current=1 s  i_L_specify=off  i_L_priority=High  i_L=0 A  i_L_nominal_specify=off  i_L_nominal_value=1  i_L_nominal_unit=A  faulted_specify=off  faulted_priority=None  faulted=0
  LDl : ee_lib/Passive/Inductor  Commented=on  l=1e-6 H  enable_L_tol=ee.enum.toleranceApplication.none  L_tol=20  tol_distribution=ee.enum.toleranceDistribution.uniform  nSigma=4  r=0 Ohm  g=1e-9 1/Ohm  enable_operating_limits=ee.enum.enable.no  operating_limit_action=ee.enum.passive.reportOpLim.warn  max_working_current=1 A  power_rating=1 W  enable_faults=ee.enum.enable.no  fault_action=simscape.enum.assert.action.none  lambdaPercent=50  k_faulted=0.9999  turnsShort=ee.enum.passive.inductor.turnsShortOption.no  openCct=ee.enum.enable.no  groundShort=ee.enum.passive.inductor.groundShortOption.no  groundShortG=0 1/Ohm  tau_fault=1e-3 s  fault_trigger=ee.enum.faults.faultTrigger.temporal  t_fault=1 s  max_permissible_voltage=100 V  n_fail_on_voltage=1  max_permissible_current=1 A  t_fail_on_current=1 s  i_L_specify=off  i_L_priority=High  i_L=0 A  i_L_nominal_specify=off  i_L_nominal_value=1  i_L_nominal_unit=A  faulted_specify=off  faulted_priority=None  faulted=0
  LDl1 : ee_lib/Passive/Inductor  Commented=on  l=1e-6 H  enable_L_tol=ee.enum.toleranceApplication.none  L_tol=20  tol_distribution=ee.enum.toleranceDistribution.uniform  nSigma=4  r=0 Ohm  g=1e-9 1/Ohm  enable_operating_limits=ee.enum.enable.no  operating_limit_action=ee.enum.passive.reportOpLim.warn  max_working_current=1 A  power_rating=1 W  enable_faults=ee.enum.enable.no  fault_action=simscape.enum.assert.action.none  lambdaPercent=50  k_faulted=0.9999  turnsShort=ee.enum.passive.inductor.turnsShortOption.no  openCct=ee.enum.enable.no  groundShort=ee.enum.passive.inductor.groundShortOption.no  groundShortG=0 1/Ohm  tau_fault=1e-3 s  fault_trigger=ee.enum.faults.faultTrigger.temporal  t_fault=1 s  max_permissible_voltage=100 V  n_fail_on_voltage=1  max_permissible_current=1 A  t_fail_on_current=1 s  i_L_specify=off  i_L_priority=High  i_L=0 A  i_L_nominal_specify=off  i_L_nominal_value=1  i_L_nominal_unit=A  faulted_specify=off  faulted_priority=None  faulted=0
  LPF4thHarmonicF_sw1 : TransferFcn  Commented=on  Numerator=2*pi*50*feNom  Denominator=[1 2*pi*50*feNom]
  LPF4thHarmonicF_sw2 : TransferFcn  Commented=on  Numerator=2*pi*1.1*f_sw  Denominator=[1 2*pi*1.1*f_sw]
  LQ : ee_lib/Passive/Inductor  Commented=on  l=1e-6 H  enable_L_tol=ee.enum.toleranceApplication.none  L_tol=20  tol_distribution=ee.enum.toleranceDistribution.uniform  nSigma=4  r=0 Ohm  g=1e-9 1/Ohm  enable_operating_limits=ee.enum.enable.no  operating_limit_action=ee.enum.passive.reportOpLim.warn  max_working_current=1 A  power_rating=1 W  enable_faults=ee.enum.enable.no  fault_action=simscape.enum.assert.action.none  lambdaPercent=50  k_faulted=0.9999  turnsShort=ee.enum.passive.inductor.turnsShortOption.no  openCct=ee.enum.enable.no  groundShort=ee.enum.passive.inductor.groundShortOption.no  groundShortG=0 1/Ohm  tau_fault=1e-3 s  fault_trigger=ee.enum.faults.faultTrigger.temporal  t_fault=1 s  max_permissible_voltage=100 V  n_fail_on_voltage=1  max_permissible_current=1 A  t_fail_on_current=1 s  i_L_specify=off  i_L_priority=High  i_L=0 A  i_L_nominal_specify=off  i_L_nominal_value=1  i_L_nominal_unit=A  faulted_specify=off  faulted_priority=None  faulted=0
  LQl : ee_lib/Passive/Inductor  Commented=on  l=1e-6 H  enable_L_tol=ee.enum.toleranceApplication.none  L_tol=20  tol_distribution=ee.enum.toleranceDistribution.uniform  nSigma=4  r=0 Ohm  g=1e-9 1/Ohm  enable_operating_limits=ee.enum.enable.no  operating_limit_action=ee.enum.passive.reportOpLim.warn  max_working_current=1 A  power_rating=1 W  enable_faults=ee.enum.enable.no  fault_action=simscape.enum.assert.action.none  lambdaPercent=50  k_faulted=0.9999  turnsShort=ee.enum.passive.inductor.turnsShortOption.no  openCct=ee.enum.enable.no  groundShort=ee.enum.passive.inductor.groundShortOption.no  groundShortG=0 1/Ohm  tau_fault=1e-3 s  fault_trigger=ee.enum.faults.faultTrigger.temporal  t_fault=1 s  max_permissible_voltage=100 V  n_fail_on_voltage=1  max_permissible_current=1 A  t_fail_on_current=1 s  i_L_specify=off  i_L_priority=High  i_L=0 A  i_L_nominal_specify=off  i_L_nominal_value=1  i_L_nominal_unit=A  faulted_specify=off  faulted_priority=None  faulted=0
  LowPassFilter2 : Subsystem  Commented=on
  MinMax Running Resettable{1,11,13,15,17} (5 alike) : simulink/Math Operations/MinMax Running Resettable  Commented=on  Function=max  vinit=0.0
  MinMax Running Resettable{2,12,14,16,18} (5 alike) : simulink/Math Operations/MinMax Running Resettable  Commented=on  Function=min  vinit=0.0
  Mux : Mux  Commented=on  Inputs=2
  Mux2 : Mux  Inputs=2
  RDC : fl_lib/Electrical/Electrical Elements/Resistor  Commented=on  R=1 Ohm  i_specify=off  i_priority=None  i=0 A  i_nominal_specify=off  i_nominal_value=1  i_nominal_unit=A  v_specify=off  v_priority=None  v=0 V  v_nominal_specify=off  v_nominal_value=1  v_nominal_unit=V
  Rcd : fl_lib/Electrical/Electrical Elements/Resistor  Commented=on  R=1 Ohm  i_specify=off  i_priority=None  i=0 A  i_nominal_specify=off  i_nominal_value=1  i_nominal_unit=A  v_specify=off  v_priority=None  v=0 V  v_nominal_specify=off  v_nominal_value=1  v_nominal_unit=V
  Rcd1 : fl_lib/Electrical/Electrical Elements/Resistor  Commented=on  R=1 Ohm  i_specify=off  i_priority=None  i=0 A  i_nominal_specify=off  i_nominal_value=1  i_nominal_unit=A  v_specify=off  v_priority=None  v=0 V  v_nominal_specify=off  v_nominal_value=1  v_nominal_unit=V
  Rcq : fl_lib/Electrical/Electrical Elements/Resistor  Commented=on  R=1 Ohm  i_specify=off  i_priority=None  i=0 A  i_nominal_specify=off  i_nominal_value=1  i_nominal_unit=A  v_specify=off  v_priority=None  v=0 V  v_nominal_specify=off  v_nominal_value=1  v_nominal_unit=V
  Rsd : fl_lib/Electrical/Electrical Elements/Resistor  Commented=on  R=1 Ohm  i_specify=off  i_priority=None  i=0 A  i_nominal_specify=off  i_nominal_value=1  i_nominal_unit=A  v_specify=off  v_priority=None  v=0 V  v_nominal_specify=off  v_nominal_value=1  v_nominal_unit=V
  Rsq : fl_lib/Electrical/Electrical Elements/Resistor  Commented=on  R=1 Ohm  i_specify=off  i_priority=None  i=0 A  i_nominal_specify=off  i_nominal_value=1  i_nominal_unit=A  v_specify=off  v_priority=None  v=0 V  v_nominal_specify=off  v_nominal_value=1  v_nominal_unit=V
  SampleWhenCarrierHasPeak1 : Subsystem  Commented=on
  Scope{4,6,8..9,11..13,15..16,18,21} (11 alike) : Scope  Commented=on
      Scope11 settings: ActiveDisplayYMinimum=-0.01675  ActiveDisplayYMaximum=0.15072
      Scope12 settings: ActiveDisplayYMinimum=9.77345  ActiveDisplayYMaximum=10.19889  DataLoggingVariableName=ScopeData13
      Scope13 settings: ActiveDisplayYMinimum=-0.48949  ActiveDisplayYMaximum=0.50621  DataLoggingVariableName=ScopeData14
      Scope15 settings: ActiveDisplayYMinimum=-6.88703  ActiveDisplayYMaximum=9.27885  DataLoggingVariableName=ScopeData2
      Scope16 settings: ActiveDisplayYMinimum=-32.33742  ActiveDisplayYMaximum=15.9505  DataLoggingVariableName=ScopeData3
      Scope18 settings: ActiveDisplayYMinimum=-0.23763  ActiveDisplayYMaximum=0.23089  DataLoggingVariableName=ScopeData15
      Scope21 settings: ActiveDisplayYMinimum=-0.24881  ActiveDisplayYMaximum=0.24881  DataLoggingVariableName=ScopeData16
      Scope4 settings: ActiveDisplayYMinimum=-0.125  ActiveDisplayYMaximum=1.125  DataLoggingVariableName=ScopeData6
      Scope6 settings: ActiveDisplayYMinimum=-9.46102  ActiveDisplayYMaximum=9.96635  DataLoggingVariableName=ScopeData8
      Scope8 settings: ActiveDisplayYMinimum=-0.125  ActiveDisplayYMaximum=1.125  DataLoggingVariableName=ScopeData10
      Scope9 settings: ActiveDisplayYMinimum=-3.55476  ActiveDisplayYMaximum=3.7414  DataLoggingVariableName=ScopeData11
  Scope14 : Scope  Commented=on  NumInputPorts=4
      settings: ActiveDisplayYMinimum=-13.23691  ActiveDisplayYMaximum=13.24713  DataLoggingVariableName=ScopeData12
  Scope{3,5,7,20} (4 alike) : Scope
      Scope20 settings: ActiveDisplayYMinimum=-41.0031  ActiveDisplayYMaximum=39.99642  DataLoggingVariableName=ScopeData4
      Scope3 settings: ActiveDisplayYMinimum=-34.62836  ActiveDisplayYMaximum=27.66497  DataLoggingVariableName=ScopeData5
      Scope5 settings: ActiveDisplayYMinimum=-0.125  ActiveDisplayYMaximum=1.125  DataLoggingVariableName=ScopeData7
      Scope7 settings: ActiveDisplayYMinimum=-1.06296  ActiveDisplayYMaximum=1.17513  DataLoggingVariableName=ScopeData9
  Second-Order Filter : eeGeneralControl/Second-Order Filter  FilterType=Low-pass  fn=feNom  Zeta=0.707  Ts=Ts  A0=0  Ph0=0  f0=0  b0=0
      settings: LibrarySourceBlock=ee_sl_lib/General Control/Second-Order Filter
  Second-Order Filter2 : eeGeneralControl/Second-Order Filter  Commented=on  FilterType=Band-pass  fn=round(mf)*feNom  Zeta=0.75  Ts=0  A0=0  Ph0=0  f0=0  b0=0
      settings: LibrarySourceBlock=ee_sl_lib/General Control/Second-Order Filter
  Second-Order Filter6 : eeGeneralControl/Second-Order Filter  Commented=on  FilterType=Low-pass  fn=round(mf)*feNom  Zeta=0.75  Ts=0  A0=0  Ph0=0  f0=0  b0=0
      settings: LibrarySourceBlock=ee_sl_lib/General Control/Second-Order Filter
  Second-Order Filter7 : eeGeneralControl/Second-Order Filter  Commented=on  FilterType=High-pass  fn=round(mf)*feNom  Zeta=0.75  Ts=0  A0=0  Ph0=0  f0=0  b0=0
      settings: LibrarySourceBlock=ee_sl_lib/General Control/Second-Order Filter
  Sine Wave11 : Sin  Commented=on  Amplitude=0.01  Frequency=4*f_sw*2*pi  SampleTime=0
  Sine Wave13 : Sin  Commented=on  Amplitude=0.1  Frequency=f_sw*2*pi  SampleTime=0
  Sine Wave3 : Sin  Commented=on  Amplitude=10  Frequency=feNom*2*pi  SampleTime=Ts
  Sine Wave4 : Sin  Commented=on  Amplitude=0.6  Frequency=100*feNom*2*pi  SampleTime=Ts
  Sine Wave7 : Sin  Commented=on  Amplitude=0.08  Frequency=f_sw*2*pi  SampleTime=0
  Sine Wave8 : Sin  Commented=on  Amplitude=0.05  Frequency=2*f_sw*2*pi  SampleTime=0
  Sine Wave9 : Sin  Commented=on  Amplitude=0.03  Frequency=3*f_sw*2*pi  SampleTime=0
  Sum3 : Sum  Commented=on  Inputs=|++
  Switch : Switch  Commented=on  Criteria=u2 > Threshold  SaturateOnIntegerOverflow=off  InputSameDT=off
  VD : ee_lib/Additional Components/SPICE Sources/DC Voltage Source  Commented=on  DC=0 V
  VD1 : ee_lib/Additional Components/SPICE Sources/DC Voltage Source  Commented=on  DC=0 V
  VQ : ee_lib/Additional Components/SPICE Sources/DC Voltage Source  Commented=on  DC=0 V
  Vector Concatenate1 : Concatenate  Commented=on  NumInputs=4  Mode=Multidimensional array
  Zero-Order Hold : ZeroOrderHold  Commented=on  SampleTime=Ts
  tag scope: RippleAmpl=global, filterCurrentA=global, rawCurrentA=global
  wires:
  From6/1 -> SampleWhenCarrierHasPeak1/Enable
  ? -> MinMax Running Resettable13/1, MinMax Running Resettable14/1
  CustomRunningAverage1/1(Mean) -> Scope15/1, Switch/1, Enabled Subsystem2/1(RippleSignal)
  Gain8/1 -> Goto12/1, Display10/1
  Enabled Subsystem3/1(Ripple) -> Gain8/1
  Zero-Order Hold/1 -> Buffer/1
  Switch/1 -> MinMax Running Resettable2/1, MinMax Running Resettable1/1
  Constant2/1 -> GreaterThan/2
  Gain6/1 -> Display8/1
  Second-Order Filter2/1 -> Scope6/1, Enabled Subsystem3/1(RippleSignal)
  Second-Order Filter/1 -> Scope3/1
  Constant4/1 -> Switch/3
  Gain9/1 -> Goto10/1, Display5/1, Vector Concatenate1/1
  Gain13/1 -> Vector Concatenate1/2, Display13/1
  GreaterThan1/1 -> Switch/2
  Enabled Subsystem1/1(Ripple) -> Gain5/1
  Constant3/1 -> GreaterThan1/2
  Gain7/1 -> Display9/1
  Clock1/1 -> GreaterThan1/1
  Enabled Subsystem2/1(Ripple) -> Gain6/1
  MinMax Running Resettable1/1 -> Add6/1
  Add6/1 -> Gain7/1
  Add8/1 -> Gain10/1
  Add10/1 -> Gain11/1
  GreaterThan/1 -> Enabled Subsystem/Enable, Scope5/1
  Gain11/1 -> Vector Concatenate1/4, Display15/1
  Gain5/1 -> Display7/1, Scope11/1
  MinMax Running Resettable18/1 -> Add10/2
  Gain4/1 -> Abs2/1
  CustomRunningAverage/1(Mean) -> [filterCurrentA], Mux2/2, Add9/2
  FFT/1 -> Gain4/1
  Gain10/1 -> Vector Concatenate1/3, Display14/1
  ? -> MinMax Running Resettable15/1, MinMax Running Resettable16/1
  Gain1/1 -> [RippleAmpl], Display6/1
  ? -> Scope16/1, Zero-Order Hold/1
  Second-Order Filter7/1 -> Second-Order Filter6/1
  MinMax Running Resettable2/1 -> Add6/2
  Add9/1 -> Scope7/1, Enabled Subsystem/1(RippleSignal)
  Vector Concatenate1/1 -> Goto11/1
  Enabled Subsystem/1(Ripple) -> Gain1/1
  MinMax Running Resettable12/1 -> Add5/2
  Demux1/1 -> Goto6/1, Second-Order Filter/1, [rawCurrentA], Mux2/1, Add9/1, CustomRunningAverage/1(In1)
  Add7/1 -> Gain13/1
  MinMax Running Resettable16/1 -> Add8/2
  Buffer/1 -> FFT/1
  Abs2/1 -> Array Plot/1
  Clock/1 -> GreaterThan/1
  MinMax Running Resettable15/1 -> Add8/1
  Gain12/1 -> Goto9/1
  Mux2/1 -> Scope20/1
  Constant11/1 -> Gain12/1
  MinMax Running Resettable14/1 -> Add7/2
  MinMax Running Resettable13/1 -> Add7/1
  MinMax Running Resettable17/1 -> Add10/1
  Add5/1 -> Gain9/1
  ? -> MinMax Running Resettable17/1, MinMax Running Resettable18/1
  MinMax Running Resettable11/1 -> Add5/1
  Second-Order Filter6/1 -> Scope9/1, Enabled Subsystem1/1(RippleSignal)
  From7/1 -> Demux2/1
  Add4/1 -> Scope14/4
  HighPassFilter3/1(Output) -> Scope14/3, Add4/2
  Sum3/1 -> HighPassFilter3/1(Input), Scope14/1, LowPassFilter2/1(Input), Add4/1
  LowPassFilter2/1(Output) -> Scope14/2
  Sine Wave3/1 -> Sum3/1
  Sine Wave4/1 -> Sum3/2
  Fund/1 -> Add2/1
  F_swHPF8/1 -> LPF4thHarmonicF_sw2/1
  LPF4thHarmonicF_sw1/1 -> Mux/2
  LPF4thHarmonicF_sw2/1 -> Scope18/1
  Sine Wave9/1 -> Add3/4
  Sine Wave13/1 -> Add3/1
  Add2/1 -> F_swHPF8/1, F_swHPF7/1, Mux/1, LPF4thHarmonicF_sw1/1
  Add3/1 -> Add2/2, Scope21/1
  F_swHPF7/1 -> Scope13/1
  Sine Wave7/1 -> Add3/2
  Mux/1 -> Scope12/1
  Sine Wave8/1 -> Add3/3
  Sine Wave11/1 -> Add3/5
  [IabcMotor] -> Demux1/1
  connections:
  Rcd/LConn1 -- Rsq/RConn1 -- LD/LConn1
  Rcd1/RConn1 -- LD1/RConn1 -- LDl1/LConn1
  RDC/RConn1 -- Rcd1/LConn1 -- LD1/LConn1
  Rcq/RConn1 -- BackEMFQ/RConn1 -- LQl/LConn1
  Rcq/LConn1 -- Rsd/RConn1 -- LQ/LConn1
  Rcd/RConn1 -- BackEMFD/LConn1 -- LDl/LConn1
  LDl1/RConn1 -- VD1/RConn1
  LDl/RConn1 -- VD/RConn1
  VQ/LConn1 -- Rsd/LConn1
  LQl/RConn1 -- VQ/RConn1
  VD1/LConn1 -- RDC/LConn1
  VD/LConn1 -- Rsq/LConn1
  BackEMFQ/LConn1 -- LQ/RConn1
  BackEMFD/RConn1 -- LD/RConn1

== system Twin_Builder/PMSM /LUTS/Usefeul/Some Tests for Filters (Useful)/CustomRunningAverage ==
  In1 : Inport
  Add2 : Sum  Inputs=+-
  Gain1 : Gain  Gain=1/(Ts)
  Integrator : Integrator
  Transport Delay : TransportDelay  DelayTime=Ts  BufferSize=2048
  Mean : Outport
  wires:
  Integrator/1 -> Add2/1, Transport Delay/1
  In1/1 -> Integrator/1
  Transport Delay/1 -> Add2/2
  Gain1/1 -> Mean/1
  Add2/1 -> Gain1/1

== system Twin_Builder/PMSM /LUTS/Usefeul/Some Tests for Filters (Useful)/CustomRunningAverage1 ==
  In1 : Inport
  Add2 : Sum  Inputs=+-
  Gain1 : Gain  Gain=1/(Ts)
  Integrator : Integrator
  Transport Delay : TransportDelay  DelayTime=Ts  BufferSize=2048
  Mean : Outport
  wires:
  Integrator/1 -> Add2/1, Transport Delay/1
  In1/1 -> Integrator/1
  Transport Delay/1 -> Add2/2
  Gain1/1 -> Mean/1
  Add2/1 -> Gain1/1

== system Twin_Builder/PMSM /LUTS/Usefeul/Some Tests for Filters (Useful)/Enabled Subsystem ==
  RippleSignal : Inport
  Enable : EnablePort
  Add1 : Sum  Inputs=+-
  Max : MinMax  Function=max  Inputs=2
  Max1 : MinMax  Inputs=2
  Memory : Memory
  Memory1 : Memory
  Ripple : Outport
  wires:
  RippleSignal/1 -> Max1/1, Max/1
  Max/1 -> Add1/1, Memory/1
  Memory/1 -> Max/2
  Max1/1 -> Add1/2, Memory1/1
  Memory1/1 -> Max1/2
  Add1/1 -> Ripple/1

== system Twin_Builder/PMSM /LUTS/Usefeul/Some Tests for Filters (Useful)/Enabled Subsystem1 ==
  RippleSignal : Inport
  Enable : EnablePort
  Add1 : Sum  Inputs=+-
  Max : MinMax  Function=max  Inputs=2
  Max1 : MinMax  Inputs=2
  Memory : Memory
  Memory1 : Memory
  Ripple : Outport
  wires:
  RippleSignal/1 -> Max1/1, Max/1
  Max/1 -> Add1/1, Memory/1
  Memory/1 -> Max/2
  Max1/1 -> Add1/2, Memory1/1
  Memory1/1 -> Max1/2
  Add1/1 -> Ripple/1

== system Twin_Builder/PMSM /LUTS/Usefeul/Some Tests for Filters (Useful)/Enabled Subsystem2 ==
  RippleSignal : Inport
  Enable : EnablePort
  Add1 : Sum  Inputs=+-
  Max : MinMax  Function=max  Inputs=2
  Max1 : MinMax  Inputs=2
  Memory : Memory
  Memory1 : Memory
  Ripple : Outport
  wires:
  RippleSignal/1 -> Max1/1, Max/1
  Max/1 -> Add1/1, Memory/1
  Memory/1 -> Max/2
  Max1/1 -> Add1/2, Memory1/1
  Memory1/1 -> Max1/2
  Add1/1 -> Ripple/1

== system Twin_Builder/PMSM /LUTS/Usefeul/Some Tests for Filters (Useful)/Enabled Subsystem3 ==
  RippleSignal : Inport
  Enable : EnablePort
  Add1 : Sum  Inputs=+-
  Max : MinMax  Function=max  Inputs=2
  Max1 : MinMax  Inputs=2
  Memory : Memory
  Memory1 : Memory
  Ripple : Outport
  wires:
  RippleSignal/1 -> Max1/1, Max/1
  Max/1 -> Add1/1, Memory/1
  Memory/1 -> Max/2
  Max1/1 -> Add1/2, Memory1/1
  Memory1/1 -> Max1/2
  Add1/1 -> Ripple/1

== system Twin_Builder/PMSM /LUTS/Usefeul/Some Tests for Filters (Useful)/HighPassFilter3 ==
  Input : Inport
  Add : Sum  Inputs=+-
  Discrete Derivative : simulink/Quick Insert/Discrete/Discrete Derivative  gainval=1  ICPrevScaledInput=0.0  OutMin=[]  OutMax=[]  OutDataType=fixdt(1, 16)  OutScaling=2^-10  DoSatur=off
  Discrete Derivative1 : simulink/Quick Insert/Discrete/Discrete Derivative  gainval=1  ICPrevScaledInput=0.0  OutMin=[]  OutMax=[]  OutDataType=fixdt(1, 16)  OutScaling=2^-10  DoSatur=off
  Gain : Gain  Gain=(100*feNom*2*pi)
  Output : Outport
  wires:
  Input/1 -> Discrete Derivative/1
  Discrete Derivative/1 -> Add/1
  Discrete Derivative1/1 -> Add/2
  Add/1 -> Gain/1
  Gain/1 -> Discrete Derivative1/1, Output/1

== system Twin_Builder/PMSM /LUTS/Usefeul/Some Tests for Filters (Useful)/LowPassFilter2 ==
  Input : Inport
  Add : Sum  Inputs=+-
  Discrete Derivative : simulink/Quick Insert/Discrete/Discrete Derivative  gainval=1/(5*feNom*2*pi)  ICPrevScaledInput=0.0  OutMin=[]  OutMax=[]  OutDataType=fixdt(1, 16)  OutScaling=2^-10  DoSatur=off
  Scope : Scope
      settings: ActiveDisplayYMinimum=-11.8504  ActiveDisplayYMaximum=11.86084  DataLoggingVariableName=ScopeData5
  Output : Outport
  wires:
  Discrete Derivative/1 -> Add/2
  Input/1 -> Add/1
  Add/1 -> Scope/1, Output/1, Discrete Derivative/1

== system Twin_Builder/PMSM /LUTS/Usefeul/Some Tests for Filters (Useful)/SampleWhenCarrierHasPeak1 ==
  theta : Inport
  Enable : EnablePort
  thetaSampled : Outport
  wires:
  theta/1 -> thetaSampled/1

== matlab function Twin_Builder/PMSM /Stop Shaft ==
  settings: updateMethod=DISCRETE
  data: Te input; TorqueNet input; Speed input; TorqueNetLim output
function TorqueNetLim = fcn(Te, TorqueNet, Speed)

TorqueNetLim = MechanicalStop(Te, TorqueNet, Speed);

== matlab function Twin_Builder/Inverter/Create VRef/Determine Common Mode Signal/DPWM1 Technique ==
  settings: updateMethod=DISCRETE  sampleTime=Ts
  data: VaRef input; Vcommon output; VbRef input; VcRef input
function Vcommon  = fcn(VaRef, VbRef, VcRef)

% Compute absolute values of the phase references
Va_abs = abs(VaRef);
Vb_abs = abs(VbRef);
Vc_abs = abs(VcRef);

% Find the maximum absolute voltage
Vmax = max([Va_abs, Vb_abs, Vc_abs]);

% Determine which phase has the max and compute Vcommon
if Va_abs == Vmax
    Vcommon = sign(VaRef) * 1.0 - VaRef;
elseif Vb_abs == Vmax
    Vcommon = sign(VbRef) * 1.0 - VbRef;
else
    Vcommon = sign(VcRef) * 1.0 - VcRef;
end
